simulink model "tb_structure_env"  (R2026b)
settings: Solver=ode3  StopTime=2  FixedStep=Ts.env  EnableMultiTasking=on
model workspace (MAT data in the model file):
  tbe.pose = [0 0 0]
  tbe.speed = 0
  tbe.use_T = 0
  tbe.T_ovr = 300
  tbe.t_ovr = 1
  tbe.use_G = 0
  tbe.G_ovr = 500
  tbe.use_soil = 0
  tbe.soil_ovr = 5
  tbe.dock_force = 0
undefined symbols (not defined in the file or in its folder): Ts
settings Model: Creator=aomar  LastModifiedBy=aomar
settings ConfigSet: Description=Shaddad fixed-step 1 ms ode3, multitasking, explicit rate transitions (arch 7, D58).
settings OptimizationCC: SimCompilerOptimization=on
settings DebuggingCC: AlgebraicLoopMsg=error  ArtificialAlgebraicLoopMsg=error  SingleTaskRateTransMsg=error  StrictBusMsg=ErrorOnBusTreatedAsVector
settings SimscapeCC: SimscapeNominalValues="[{\"value\":\"1\",\"unit\":\"A\"},{\"value\":\"1\",\"unit\":\"bar\"},{\"value\":\"1\",\"unit\":\"cm^2\"},{\"value\":\"1\",\"unit\":\"cm^3/s\"},{\"value\":\"1\",\"unit\":\"kJ/kg\"},{\"value\":\"1\",\"unit\":\"kW\"},{\"value\":\"1\",\"unit\":\"l\"},{\"value\":\"1\",\"unit\":\"N\"},{\"value\":\"1\",\"unit\":\"N*m\"},{\"value\":\"1\",\"unit\":\"V\"},{\"value\":\"0.001\",\"unit\":\"Wb\"}]"  SimscapeNormalizeSystem=off  SimscapeUseEnergyAccounting=off

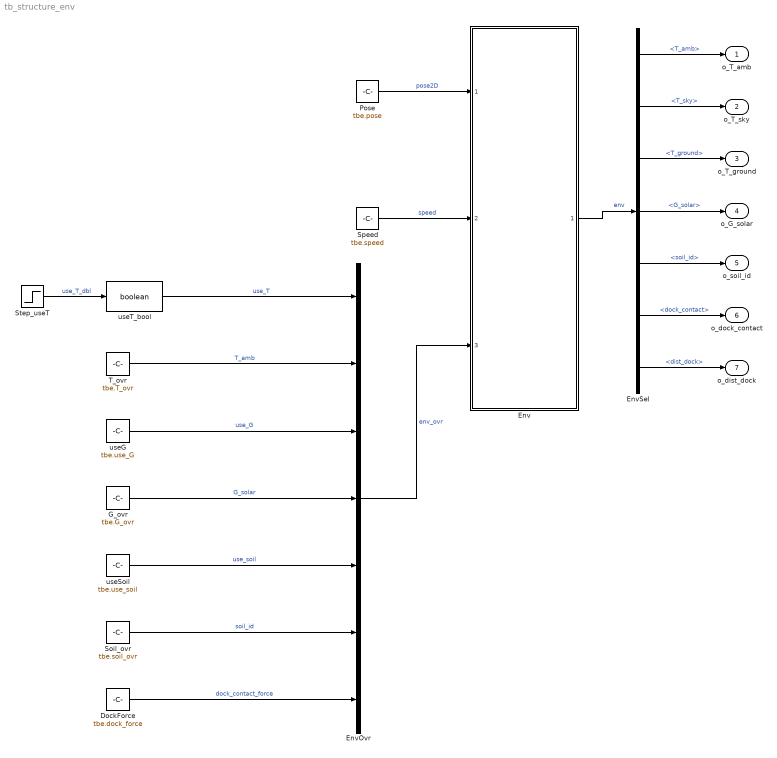
== system tb_structure_env ==
  DockForce : Constant  Value=tbe.dock_force  OutDataTypeStr=boolean  SampleTime=Ts.env
  Env : Subsystem  ReferencedSubsystem=structure_env
  EnvOvr : BusCreator  Inputs=7  OutDataTypeStr=Bus: Bus_EnvOverride  NonVirtualBus=on
  EnvSel : BusSelector  OutputSignals=T_amb,T_sky,T_ground,G_solar,soil_id,dock_contact,dist_dock
  G_ovr : Constant  Value=tbe.G_ovr  SampleTime=Ts.env
  Pose : Constant  Value=tbe.pose  SampleTime=0
  Soil_ovr : Constant  Value=tbe.soil_ovr  OutDataTypeStr=uint8  SampleTime=Ts.env
  Speed : Constant  Value=tbe.speed  SampleTime=0
  Step_useT : Step  Time=tbe.t_ovr  FinalValue=tbe.use_T  SampleTime=Ts.env
  T_ovr : Constant  Value=tbe.T_ovr  SampleTime=Ts.env
  useG : Constant  Value=tbe.use_G  OutDataTypeStr=boolean  SampleTime=Ts.env
  useSoil : Constant  Value=tbe.use_soil  OutDataTypeStr=boolean  SampleTime=Ts.env
  useT_bool : DataTypeConversion  OutDataTypeStr=boolean  SaturateOnIntegerOverflow=off  RndMeth=Floor
  o_T_amb : Outport
  o_T_sky : Outport  Port=2
  o_T_ground : Outport  Port=3
  o_G_solar : Outport  Port=4
  o_soil_id : Outport  Port=5
  o_dock_contact : Outport  Port=6
  o_dist_dock : Outport  Port=7
  wires:
  Step_useT/1 -> useT_bool/1  "use_T_dbl"
  T_ovr/1 -> EnvOvr/2  "T_amb"
  useG/1 -> EnvOvr/3  "use_G"
  G_ovr/1 -> EnvOvr/4  "G_solar"
  useSoil/1 -> EnvOvr/5  "use_soil"
  Soil_ovr/1 -> EnvOvr/6  "soil_id"
  DockForce/1 -> EnvOvr/7  "dock_contact_force"
  useT_bool/1 -> EnvOvr/1  "use_T"
  EnvOvr/1 -> Env/3  "env_ovr"
  Pose/1 -> Env/1  "pose2D"
  Speed/1 -> Env/2  "speed"
  Env/1 -> EnvSel/1  "env"
  EnvSel/1 -> o_T_amb/1  "<T_amb>"
  EnvSel/2 -> o_T_sky/1  "<T_sky>"
  EnvSel/3 -> o_T_ground/1  "<T_ground>"
  EnvSel/4 -> o_G_solar/1  "<G_solar>"
  EnvSel/5 -> o_soil_id/1  "<soil_id>"
  EnvSel/6 -> o_dock_contact/1  "<dock_contact>"
  EnvSel/7 -> o_dist_dock/1  "<dist_dock>"
